simulink model "observerSimulation"  (R2016a)
settings: Solver=VariableStepAuto  StartTime=0.0  StopTime=15.0  RelTol=1e-6
undefined symbols (not defined in the file): C, gain1, J, L, lambda, N, sys, V, z0
libraries: cstblocks x1
settings Model: Creator=Muwahida  LastModifiedBy=Muwahida

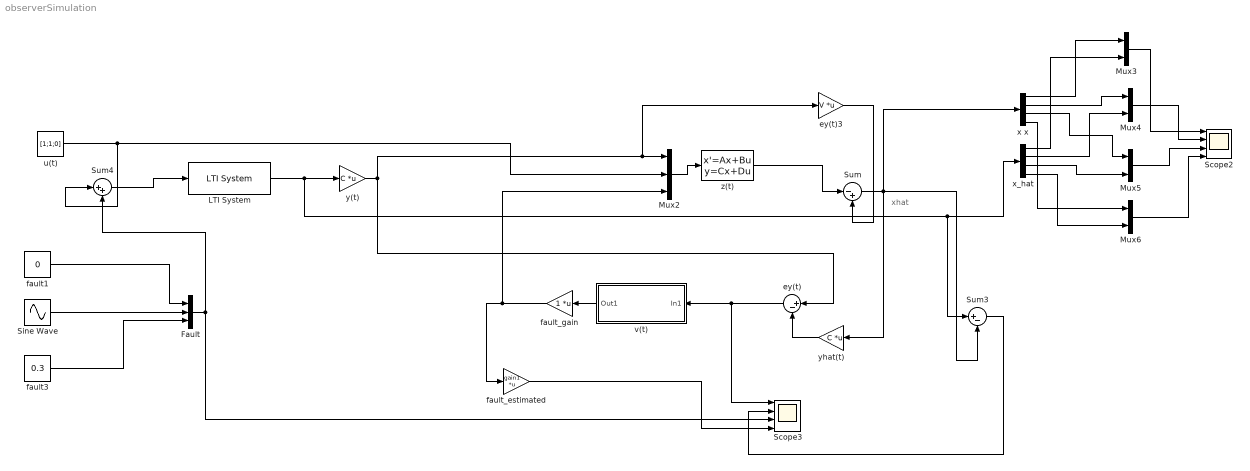
== system observerSimulation ==
  note: xhat
  Fault : Mux  Inputs=3
  LTI System : cstblocks/LTI System  sys=tf(sys)  IC=[]
  Mux2 : Mux  Inputs=3
  Mux{3..6} (4 alike) : Mux  Inputs=2
  Scope2 : Scope  NumInputPorts=4
  Scope3 : Scope  NumInputPorts=4
  Sine Wave : Sin  Amplitude=0.1  SampleTime=0
  Sum : Sum  Inputs=|-+
  Sum3 : Sum  Inputs=|+-
  Sum4 : Sum  Inputs=|++
  ey(t) : Sum  Inputs=|+-
  ey(t)3 : Gain  Gain=V  Multiplication=Matrix(K*u)
  fault1 : Constant  Value=0
  fault3 : Constant  Value=0.3
  fault_estimated : Gain  Gain=gain1  Multiplication=Matrix(K*u)
  fault_gain : Gain  Multiplication=Matrix(K*u)
  u(t) : Constant  Value=[1;1;0]
  v(t) : Subsystem
  x x : Demux  Outputs=n
  x_hat : Demux  Outputs=n
  y(t) : Gain  Gain=C  Multiplication=Matrix(K*u)
  yhat(t) : Gain  Gain=C  Multiplication=Matrix(K*u)
  z(t) : StateSpace  A=N  B="[L  J -lambda]"  C=eye(4)  D=zeros(4,9)  X0=z0
  wires:
  u(t)/1 -> Mux2/2, Sum4/1
  Mux2/1 -> z(t)/1
  z(t)/1 -> Sum/1
  y(t)/1 -> ey(t)3/1, Mux2/1, ey(t)/1
  LTI System/1 -> x_hat/1, Sum3/1, y(t)/1
  Sum/1 -> x x/1, Sum3/2, yhat(t)/1
  fault1/1 -> Fault/1
  Sum4/1 -> LTI System/1
  ey(t)3/1 -> Sum/2
  yhat(t)/1 -> ey(t)/2
  ey(t)/1 -> Scope3/1, v(t)/1(In1)
  v(t)/1(Out1) -> fault_gain/1
  Sum3/1 -> Scope3/2
  fault3/1 -> Fault/3
  x x/1 -> Mux3/1
  x_hat/1 -> Mux3/2
  x x/2 -> Mux4/1
  x_hat/2 -> Mux4/2
  x x/3 -> Mux5/1
  x_hat/3 -> Mux5/2
  x x/4 -> Mux6/1
  x_hat/4 -> Mux6/2
  Mux3/1 -> Scope2/1
  Mux4/1 -> Scope2/2
  Mux5/1 -> Scope2/3
  Mux6/1 -> Scope2/4
  Fault/1 -> Scope3/3, Sum4/2
  fault_estimated/1 -> Scope3/4
  Sine Wave/1 -> Fault/2
  fault_gain/1 -> Mux2/3, fault_estimated/1

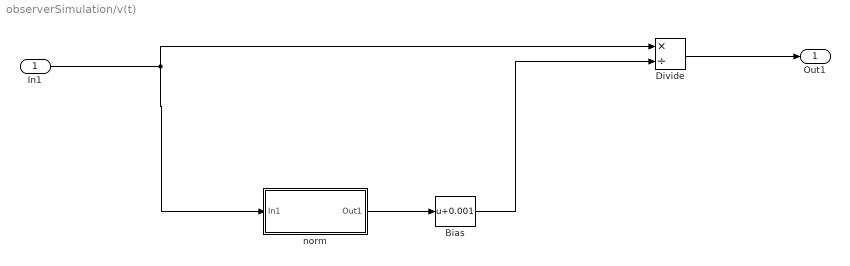
== system observerSimulation/v(t) ==
  In1 : Inport
  Bias : Bias  Bias=0.001
  Divide : Product  Inputs=*/
  norm : Subsystem
  Out1 : Outport
  wires:
  In1/1 -> norm/1(In1), Divide/1
  norm/1(Out1) -> Bias/1
  Bias/1 -> Divide/2
  Divide/1 -> Out1/1

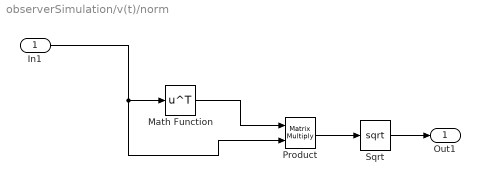
== system observerSimulation/v(t)/norm ==
  In1 : Inport
  Math Function : Math  Operator=transpose  SaturateOnIntegerOverflow=on
  Product : Product  Multiplication=Matrix(*)
  Sqrt : Sqrt  SaturateOnIntegerOverflow=on
  Out1 : Outport
  wires:
  In1/1 -> Product/2, Math Function/1
  Product/1 -> Sqrt/1
  Sqrt/1 -> Out1/1
  Math Function/1 -> Product/1
